simulink subsystem "Subsys_GFormConv_OuterCtrl_VSM"  (R2022b)
settings: Solver=VariableStepAuto  StartTime=0.0  StopTime=10.0  RelTol=1e-3
model mask{f_n=50, H=0.1, K_d=40, K=20, s_droop_QV=0.1, T_Q=0.2, T_s_ctrl=1e-3, T_s_PWM_meas=1e-4}
  mask prompts: f_n "Nominal Frequency [Hz]"; H "Virtual inertia [s]"; K_d "Damping constant K_d [pu]"; K "Droop constant K (dT/df) [pu]"; s_droop_QV "Droop constant kQ (dV[pu]/dQ[pu])"; T_Q "PT1 time constant QV-loop T_Q [s]"; T_s_ctrl "Controller sample time [s]"; T_s_PWM_meas "PWM and measurements sample time [s]"
undefined symbols (not defined in the file): alpha_LPF_Q, DiscIntNeverNeededParam
libraries: simulink x2
settings Model: Creator=winkens  LastModifiedBy=winkens
settings SolverCC: AlgebraicLoopSolver=TrustRegion
settings DebuggingCC: UnconnectedInputMsg=warning  UnconnectedOutputMsg=warning  UnconnectedLineMsg=warning  SFMachineParentedDataDiag=warning
settings ModelReferenceCC: EnableRefExpFcnMdlSchedulingChecks=on
settings RTWCC: DLArmComputeVersion=19.05

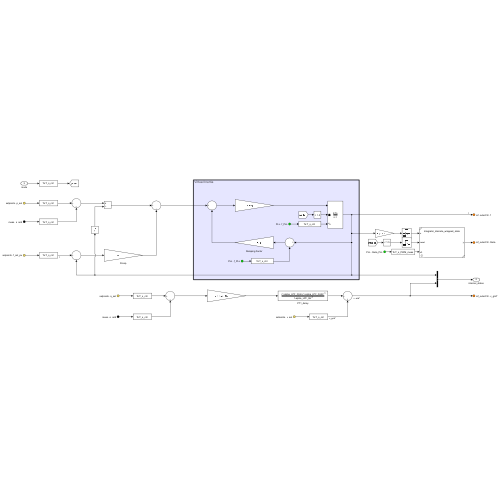
[thumbnail: Simulink's stored preview of the top-level diagram]
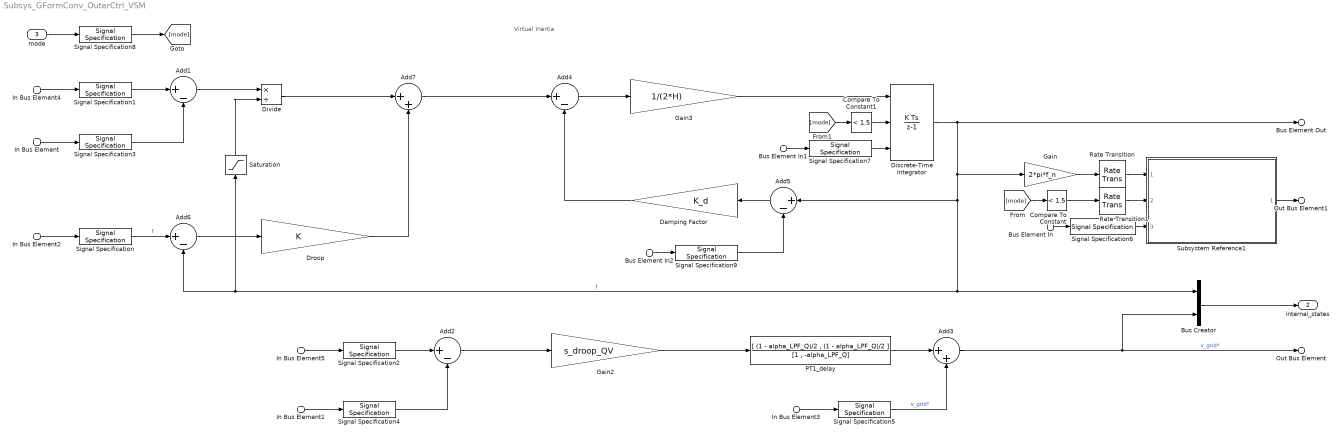
== system Subsys_GFormConv_OuterCtrl_VSM ==
  note: Virtual Inertia
  In Bus Element : Inport  PortName=meas  Element=p_grid
  In Bus Element1 : Inport  PortName=meas  Element=q_grid
  In Bus Element2 : Inport  Port=2  PortName=setpoints  Element=f_set_pu
  In Bus Element3 : Inport  Port=2  PortName=setpoints  Element=v_set
  In Bus Element4 : Inport  Port=2  PortName=setpoints  Element=p_set
  In Bus Element5 : Inport  Port=2  PortName=setpoints  Element=q_set
  mode : Inport  Port=3
  Bus Element In : Inport  Port=4  PortName=PLL  Element=theta_PLL
  Bus Element In1 : Inport  Port=4  PortName=PLL  Element=f_PLL
  Bus Element In2 : Inport  Port=4  PortName=PLL  Element=f_PLL
  Add{1..2,4..6} (5 alike) : Sum  Inputs=|+-
  Add3 : Sum  Inputs=|++
  Add7 : Sum  Inputs=|++
  Bus Creator : BusCreator  Inputs=2
  Compare To Constant : simulink/Logic and Bit Operations/Compare To Constant  relop=<  const=1.5  OutDataTypeStr=boolean
  Compare To Constant1 : simulink/Logic and Bit Operations/Compare To Constant  relop=<  const=1.5  OutDataTypeStr=boolean
  Damping Factor : Gain  Gain=K_d
  Discrete-Time Integrator : DiscreteIntegrator  ExternalReset=sampled level  InitialConditionSource=external  InitialCondition=1  SampleTime=T_s_ctrl  ICPrevOutput=DiscIntNeverNeededParam  ICPrevScaledInput=DiscIntNeverNeededParam
  Divide : Product  Inputs=*/
  Droop : Gain  Gain=K
  Gain : Gain  Gain=2*pi*f_n
  Gain2 : Gain  Gain=s_droop_QV
  Gain3 : Gain  Gain=1/(2*H)
  PT1_delay : DiscreteFilter  Numerator=[ (1 - alpha_LPF_Q)/2 , (1 - alpha_LPF_Q)/2 ]  Denominator=[1 , -alpha_LPF_Q]  SampleTime=T_s_ctrl
  Rate Transition : RateTransition  Deterministic=off  OutPortSampleTime=T_s_PWM_meas
  Rate Transition1 : RateTransition  Deterministic=off  OutPortSampleTime=T_s_PWM_meas
  Saturation : Saturate  UpperLimit=inf  LowerLimit=0.5
  Signal Specification{,1..5,7..9} (9 alike) : SignalSpecification  SampleTime=T_s_ctrl
  Signal Specification6 : SignalSpecification  SampleTime=T_s_PWM_meas
  Subsystem Reference1 : Subsystem  ReferencedSubsystem=Integrator_discrete_wrapped_state  WrappedStateUpperValue=2*pi  WrappedStateLowerValue=0  x_0=0  T_s=T_s_PWM_meas
  Out Bus Element1 : Outport  PortName=ref_outerCtrl  Element=theta
  Bus Element Out : Outport  PortName=ref_outerCtrl  Element=f
  Out Bus Element : Outport  PortName=ref_outerCtrl  Element=v_grid*
  internal_states : Outport  Port=2
  wires:
  Rate Transition1/1 -> Subsystem Reference1/2
  Rate Transition/1 -> Subsystem Reference1/1
  Signal Specification6/1 -> Subsystem Reference1/3
  Add3/1 -> Out Bus Element/1, Bus Creator/2  "v_grid*"
  Discrete-Time Integrator/1 -> Bus Element Out/1, Add6/2, Saturation/1, Bus Creator/1, Add5/1, Gain/1  "f"
  Subsystem Reference1/1 -> Out Bus Element1/1
  Bus Element In/1 -> Signal Specification6/1
  Gain/1 -> Rate Transition/1
  Bus Creator/1 -> internal_states/1
  Compare To Constant/1 -> Rate Transition1/1
  In Bus Element1/1 -> Signal Specification4/1
  In Bus Element5/1 -> Signal Specification2/1
  In Bus Element4/1 -> Signal Specification1/1
  In Bus Element/1 -> Signal Specification3/1
  In Bus Element2/1 -> Signal Specification/1
  In Bus Element3/1 -> Signal Specification5/1
  Add2/1 -> Gain2/1
  Gain2/1 -> PT1_delay/1
  PT1_delay/1 -> Add3/1
  Signal Specification5/1 -> Add3/2  "v_grid*"
  Signal Specification2/1 -> Add2/1
  Signal Specification4/1 -> Add2/2
  Signal Specification1/1 -> Add1/1
  Signal Specification3/1 -> Add1/2
  Signal Specification/1 -> Add6/1  "f"
  Add5/1 -> Damping Factor/1
  Damping Factor/1 -> Add4/2
  Add4/1 -> Gain3/1
  Gain3/1 -> Discrete-Time Integrator/1
  Bus Element In1/1 -> Signal Specification7/1
  mode/1 -> Signal Specification8/1
  [mode] -> Compare To Constant/1
  Compare To Constant1/1 -> Discrete-Time Integrator/2
  [mode] -> Compare To Constant1/1
  Signal Specification8/1 -> [mode]
  Signal Specification7/1 -> Discrete-Time Integrator/3
  Bus Element In2/1 -> Signal Specification9/1
  Signal Specification9/1 -> Add5/2
  Add7/1 -> Add4/1
  Add6/1 -> Droop/1
  Add1/1 -> Divide/1
  Divide/1 -> Add7/1
  Droop/1 -> Add7/2
  Saturation/1 -> Divide/2
